simulink model "MPC3d"  (R2024b)
settings: Solver=VariableStepAuto  StartTime=0.0  StopTime=10.0  RelTol=1e-3
values from neighbouring files (symbols this model uses):
  dis_sys = c2d(linear_sys, Ts, 'zoh')    [MPC.m]    (also in mpc3D.m = c2d(sys, Ts, 'zoh'))
libraries: mpclib x1
settings Model: Creator=xsixsipas  LastModifiedBy=xsixsipas

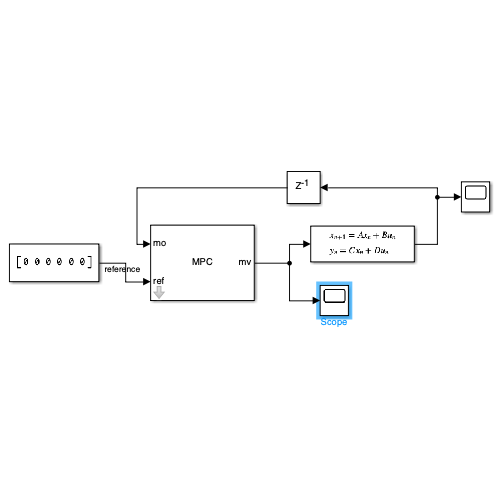
[thumbnail: Simulink's stored preview of the top-level diagram]
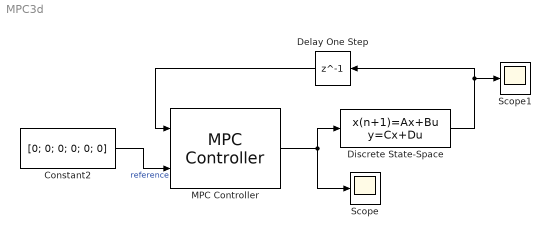
== system MPC3d ==
  Constant2 : Constant  Value=[0; 0; 0; 0; 0; 0]
  Delay One Step : Delay  DelayLength=1
  Discrete State-Space : DiscreteStateSpace  A=dis_sys.A  B=dis_sys.B  C=dis_sys.C  D=dis_sys.D  InitialCondition="[pi/6  pi/12 0 0 0 0]"  SampleTime=-1
  MPC Controller : mpclib/MPC Controller  SCDEnableBlockLinearizationSpecification=on  mpcobj=mpcobj  x0=Init_cond  is_multiple=0  enable_value=0  return_u0=off  updateMPCinCallerWorkspace=on  md_inport=off  mv_inport=off  uref_inport=off  return_cost=off  return_mvseq=off  return_qpstatus=off  return_xseq=off  return_state=off  return_ovseq=off  state_inport=off  umin_inport=off  umax_inport=off  ymin_inport=off  ymax_inport=off  cc_inport=off  ywt_inport=off  uwt_inport=off  duwt_inport=off  rhoeps_inport=off  pm_inport=off  MaximumP=10  HorizonChoice=FixedHorizon  n_ts=0.01  n_p=100  n_mv=3  n_md=0  n_ud=0  n_mo=6  n_uo=0  BlockDataType=double  SampleTimeInherited=off  switch_inport=off
  Scope : Scope
  Scope1 : Scope
  wires:
  Constant2/1 -> MPC Controller/2  "reference"
  MPC Controller/1 -> Discrete State-Space/1, Scope/1
  Discrete State-Space/1 -> Scope1/1, Delay One Step/1
  Delay One Step/1 -> MPC Controller/1
